simulink model "cktfyp"  (R2026b)
settings: Solver=VariableStepAuto  StopTime=1
undefined symbols (not defined in the file or in its folder): sim_Iload, sim_pulse_period, sim_t_fault, sim_Vdc
libraries: fl_lib x7, nesl_utility x5, ee_lib x2, simulink x1
settings Model: Creator=ASUS  LastModifiedBy=ASUS
settings SimscapeCC: SimscapeLogType=all  SimscapeNominalValues="[{\"value\":\"1\",\"unit\":\"A\"},{\"value\":\"1\",\"unit\":\"bar\"},{\"value\":\"1\",\"unit\":\"cm^2\"},{\"value\":\"1\",\"unit\":\"cm^3/s\"},{\"value\":\"1\",\"unit\":\"kJ/kg\"},{\"value\":\"1\",\"unit\":\"kW\"},{\"value\":\"1\",\"unit\":\"l\"},{\"value\":\"1\",\"unit\":\"N\"},{\"value\":\"1\",\"unit\":\"N*m\"},{\"value\":\"1\",\"unit\":\"V\"},{\"value\":\"0.001\",\"unit\":\"Wb\"}]"  SimscapeUseEnergyAccounting=off

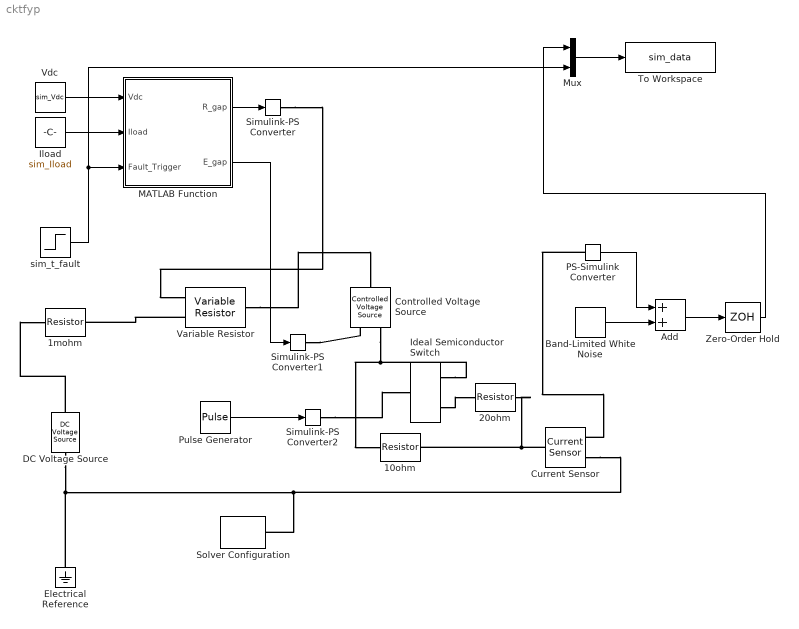
== system cktfyp ==
  10ohm : fl_lib/Electrical/Electrical Elements/Resistor  R=10 Ohm  i_specify=off  i_priority=None  i=0 A  i_nominal_specify=off  i_nominal_value=1  i_nominal_unit=A  v_specify=off  v_priority=None  v=0 V  v_nominal_specify=off  v_nominal_value=1  v_nominal_unit=V
  1mohm : fl_lib/Electrical/Electrical Elements/Resistor  R=0.01 Ohm  i_specify=off  i_priority=None  i=0 A  i_nominal_specify=off  i_nominal_value=1  i_nominal_unit=A  v_specify=off  v_priority=None  v=0 V  v_nominal_specify=off  v_nominal_value=1  v_nominal_unit=V
  20ohm : fl_lib/Electrical/Electrical Elements/Resistor  R=20 Ohm  i_specify=off  i_priority=None  i=0 A  i_nominal_specify=off  i_nominal_value=1  i_nominal_unit=A  v_specify=off  v_priority=None  v=0 V  v_nominal_specify=off  v_nominal_value=1  v_nominal_unit=V
  Add : Sum
  Band-Limited White Noise : simulink/Sources/Band-Limited White Noise  Cov=1e-5  Ts=6.25e-5  seed=[23341]
  Controlled Voltage Source : fl_lib/Electrical/Electrical Sources/Controlled Voltage Source
  Current Sensor : fl_lib/Electrical/Electrical Sensors/Current Sensor
  DC Voltage Source : ee_lib/Additional Components/SPICE Sources/DC Voltage Source  DC=50 V
  Electrical Reference : fl_lib/Electrical/Electrical Elements/Electrical Reference
  Ideal Semiconductor Switch : ee_lib/Semiconductors & Converters/Ideal Semiconductor Switch  port_option=ee.enum.controlport.ps  Ron=0.001 Ohm  Goff=1e-6 1/Ohm  Vth=0.5 V  diode_param=ee.enum.semiconductors.protectionDiode.external  diode_Vf=0.8 V  diode_Ron=0.001 Ohm  diode_Goff=1e-5 1/Ohm  diode_C=50e-9 F  diode_iRM=-235 A  diode_iF=300 A  diode_idot=-50 A/us  diode_trr_param=ee.enum.converters.diodetrr.trr_factor  diode_trr_factor=3  diode_trr=15 us  diode_Qrr=1500 s*uA
  Iload : Constant  Value=sim_Iload
  MATLAB Function : MATLAB Function  TreatAsAtomicUnit=on
  Mux : Mux  Inputs=2
  PS-Simulink Converter : nesl_utility/PS-Simulink Converter  PhysicalDomain=network_engine_domain  SubClassName=ps_output  LeftPortType=input  RightPortType=output  PseudoPeriodic=off  Frequencies=[]  VectorFormat=inherit  Unit=inherit  AffineConversion=off
  Pulse Generator : DiscretePulseGenerator  PulseType=Time based  Period=sim_pulse_period  PulseWidth=50
  Simulink-PS Converter : nesl_utility/Simulink-PS Converter  PhysicalDomain=network_engine_domain  SubClassName=ps_input  LeftPortType=input  RightPortType=output  PseudoPeriodic=off  Frequencies=[]  NoiseDistribution=none  NoiseParameters=[]  Unit=1  AffineConversion=off  FilteringAndDerivatives=provide  SimscapeFilterOrder=1  InputFilterTimeConstant=0.001  UdotUserProvided=0
  Simulink-PS Converter1 : nesl_utility/Simulink-PS Converter  PhysicalDomain=network_engine_domain  SubClassName=ps_input  LeftPortType=input  RightPortType=output  PseudoPeriodic=off  Frequencies=[]  NoiseDistribution=none  NoiseParameters=[]  Unit=1  AffineConversion=off  FilteringAndDerivatives=provide  SimscapeFilterOrder=1  InputFilterTimeConstant=0.001  UdotUserProvided=0
  Simulink-PS Converter2 : nesl_utility/Simulink-PS Converter  PhysicalDomain=network_engine_domain  SubClassName=ps_input  LeftPortType=input  RightPortType=output  PseudoPeriodic=off  Frequencies=[]  NoiseDistribution=none  NoiseParameters=[]  Unit=1  AffineConversion=off  FilteringAndDerivatives=provide  SimscapeFilterOrder=1  InputFilterTimeConstant=0.001  UdotUserProvided=0
  Solver Configuration : nesl_utility/Solver Configuration  PhysicalDomain=network_engine_domain  SubClassName=solver  LeftPortType=input  RightPortType=generic  Tones=[]  Harmonics=[]  SimulateNoise=off  Profile=off  UseLocalSampling=off  EnableSwitchedLinearOptims=on  FrequencyDomain=off  UseCCode=off  RelTol=0.001  AbsTol=0.001  MinStep=1e-09  ToWorkspace=off  RevertToSquareIcSolve=off  NumHomotopyIterations=100  PhasorMode=off  PhasorModeNumHarmonics=1  ConsistencySolver=NEWTON_XTOL_AFTER_FTOL  CanonicalOrdering=CANONICAL  OptimizeIntermediates=OPTIMIZED  MulticoreSolverChoice=BACKWARD_EULER  IndexReductionMethod=DerivativeReplacement  DoDC=off  ResidualTolerance=1e-09  ConsistencyTolSource=GLOBAL  ConsistencyAbsTol=0.001  ConsistencyRelTol=0.001  ConsistencyTolFactor=0.001  UseLocalSolver=on  LocalSolverChoice=NE_BACKWARD_EULER_ADVANCER  ResolveIndetEquations=on  FunctionEvalNumThread=1  LocalSolverSampleTime=1e-5  DoFixedCost=off  MaxNonlinIter=3  MaxModeIter=2  ComputeImpulses=off  ImpulseIterations=2  LinearAlgebra=auto  LinearAlgebraNumThread=0  EquationFormulation=NE_TIME_EF  DelaysMemoryBudget=1024  AutomaticFiltering=on  FilteringTimeConstant=0.001  PartitionStorageMethod=AS_NEEDED  PartitionMemoryBudget=1024  PartitionMethod=BALANCED  MultibodyUseLocalSolver=off  MultibodyLocalSolverChoice=ODE1  MultibodyLocalSolverSampleTime=0.001
  To Workspace : ToWorkspace  VariableName=sim_data  SampleTime=-1
  Variable Resistor : fl_lib/Electrical/Electrical Elements/Variable Resistor  Rmin=0 Ohm  thermalEnable=false  thermal_mass=1 J/K  i_specify=off  i_priority=None  i=0 A  i_nominal_specify=off  i_nominal_value=1  i_nominal_unit=A  v_specify=off  v_priority=None  v=0 V  v_nominal_specify=off  v_nominal_value=1  v_nominal_unit=V  T_specify=off  T_priority=None  T=300 K  T_nominal_specify=off  T_nominal_value=1  T_nominal_unit=K
  Vdc : Constant  Value=sim_Vdc
  Zero-Order Hold : ZeroOrderHold  SampleTime=6.25e-5
  sim_t_fault : Step  Time=sim_t_fault  SampleTime=0
  wires:
  MATLAB Function/1(R_gap) -> Simulink-PS Converter/1
  MATLAB Function/2(E_gap) -> Simulink-PS Converter1/1
  Vdc/1 -> MATLAB Function/1(Vdc)
  Iload/1 -> MATLAB Function/2(Iload)
  sim_t_fault/1 -> Mux/2, MATLAB Function/3(Fault_Trigger)
  Zero-Order Hold/1 -> Mux/1
  Mux/1 -> To Workspace/1
  Pulse Generator/1 -> Simulink-PS Converter2/1
  Band-Limited White Noise/1 -> Add/2
  Add/1 -> Zero-Order Hold/1
  PS-Simulink Converter/1 -> Add/1
  connections:
  Electrical Reference/LConn1 -- DC Voltage Source/RConn1 -- Current Sensor/RConn2 -- Solver Configuration/RConn1
  DC Voltage Source/LConn1 -- 1mohm/LConn1
  Current Sensor/LConn1 -- 10ohm/RConn1 -- 20ohm/RConn1
  PS-Simulink Converter/LConn1 -- Current Sensor/RConn1
  Variable Resistor/LConn2 -- 1mohm/RConn1
  Variable Resistor/RConn1 -- Controlled Voltage Source/LConn1
  Controlled Voltage Source/RConn2 -- Ideal Semiconductor Switch/RConn1 -- 10ohm/LConn1
  Simulink-PS Converter/RConn1 -- Variable Resistor/LConn1
  Simulink-PS Converter1/RConn1 -- Controlled Voltage Source/RConn1
  Ideal Semiconductor Switch/RConn2 -- 20ohm/LConn1
  Simulink-PS Converter2/RConn1 -- Ideal Semiconductor Switch/LConn1

== matlab function cktfyp/MATLAB Function ==
  data: Vdc input; R_gap output; Iload input; Fault_Trigger input; E_gap output
function [R_gap, E_gap] = fcn(Vdc, Iload, Fault_Trigger)
if Fault_Trigger == 1
    % ACTIVE ARC: Force q into the high-resistance burning zone (0.7 to 0.9)
    % This creates a massive, visible current drop AND high-frequency noise
    q = 0.7 + (0.2 * rand()); 
else
    % NORMAL: Contacts are completely closed
    q = 0;
end

% Calculate alpha dynamically based on closed resistance (0.001 ohms)
alpha = -0.5 * log((0.001 * Iload) / Vdc);

% Calculate Arc Resistance
R_gap = (Vdc / Iload) * exp(2 * alpha * (q - 1));

% Calculate Arc Voltage (EMF)
a = 0.01; 
b = 0.005; 
lambda = 100; 
x_gap = q * 1.5; 
E_gap = 0.5 * (a + b * x_gap) * (tanh(lambda * q) - tanh(lambda * (q - 1)));
end
